simulink model "Aero_basic_tests"  (R2025a)
settings: Solver=ode1  StartTime=0.0  StopTime=240  FixedStep=0.002  RelTol=1e-3  EnableMultiTasking=on
undefined symbols (not defined in the file or in its folder): HIL, repelem
libraries: quarc_library x5, simulink x2
settings Model: SimulationMode=external  ExtModeTrigDuration=5000  Creator=MLevis  LastModifiedBy=e82540u
settings SolverCC: AlgebraicLoopSolver=TrustRegion  PositivePriorityOrder=on
settings DataIOCC: LimitDataPoints=on  SaveFormat=Array  ReturnWorkspaceOutputs=off
settings DebuggingCC: SolverPrmCheckMsg=warning  UnconnectedInputMsg=warning  UnconnectedOutputMsg=warning  UnconnectedLineMsg=warning  SFUnexpectedBacktrackingDiag=warning  SFNoUnconditionalDefaultTransitionDiag=warning  SFExecutionAtInitializationDiag=none  ArithmeticOperatorsInVariantConditions=warning
settings ModelReferenceCC: PropagateSignalLabelsOutOfModel=off
settings SFSimCC: SimUseLocalCustomCode=off  CustomCodeUndefinedFunction=UseInterfaceOnly
settings RTWCC: SystemTargetFile=quarc_win64.tlc  TemplateMakefile=quarc_default_tmf  RTWUseLocalCustomCode=off  Toolchain=QUARC win64 | nmake (64-bit Windows)  BuildConfiguration=Faster Runs  GPUComputeCapability=3.5  Description=QUARC Win64 Target Using Toolchain
settings CodeAppCC: StateflowObjectComments=on
settings STFCustomTargetCC: SystemTargetFile=quarc_win64.tlc  MultiwordLength=2048.0  DynamicStringBufferSize=256.0  ConcurrentExecutionCompliant=on  UseToolchainInfoCompliant=on
settings GRTTargetCC: ExtMode=on  ExtModeMexFile=quarc_comm  TargetLangStandard=C89/C90 (ANSI)  ParMdlRefBuildCompliant=off  CompOptLevelCompliant=off  CombineOutputUpdateFcns=off  MatFileLogging=off  CPPClassGenCompliant=off  GRTInterface=on
settings ConfigComp: CovMetricSettings=dw  CovSaveCumulativeToWorkspaceVar=on  CovSaveSingleToWorkspaceVar=on  CovExternalEMLEnable=off  CovSFcnEnable=off

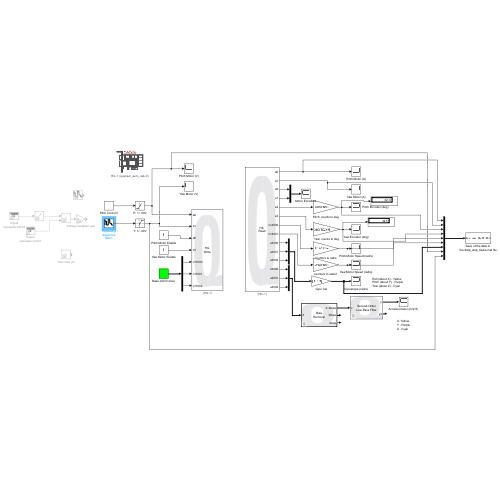
[thumbnail: Simulink's stored preview of the top-level diagram]
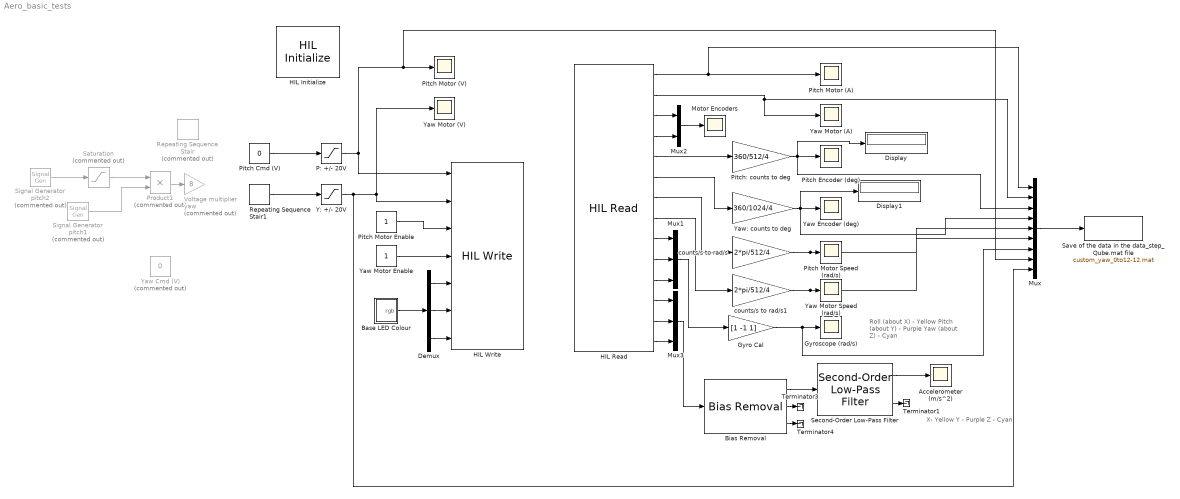
== system Aero_basic_tests ==
  note: Roll (about X) - Yellow
      | Pitch (about Y) - Purple
      | Yaw (about Z) - Cyan
  note: X- Yellow
      | Y - Purple
      | Z - Cyan
  Accelerometer (m/s^2) : Scope
      settings: DataLoggingVariableName=ScopeData10  DataLoggingSaveFormat=Array
  Base LED Colour : Subsystem  mask(Color Constant){color=[0 1 0]}
      mask help: Outputs a constant RGB color value.
      mask init:
      | rgb = get_param(gcbh, 'color');
      | if numel(color) ~= 3
      |     rgb = [0 0 0];
      | end
      | set_param(gcbh, 'MaskDisplay', ['patch([-0.02 -0.02 1.02 1.02], [-0.02 1.02 1.02 -0.02], ', rgb, ');']);
      settings: OpenFcn=color_constant_properties('CurrentBlock', gcbh);
      mask Help: web(qc_get_block_help_path(gcb), '-helpbrowser');
      mask Display: patch([-0.02 -0.02 1.02 1.02], [-0.02 1.02 1.02 -0.02], [0 1 0]);
  Bias Removal : quarc_library/Discrete/Bias Removal  start_time=0  end_time=0.1  switch_id=0  sample_time=qc_get_step_size
      settings: SourceProductName=QUARC Targets
  Demux : Demux  Outputs=3
  Display : Display
      settings: Decimation=20
  Display1 : Display
      settings: Decimation=20
  Gyro Cal : Gain  Gain=[1 -1 1]
  Gyroscope (rad/s) : Scope
      settings: TimeSpan=10  ActiveDisplayYMinimum=-2  ActiveDisplayYMaximum=2  DataLoggingVariableName=ScopeData9  DataLoggingSaveFormat=Array
  HIL Initialize : quarc_library/Data Acquisition/Generic/Configuration/HIL Initialize  Priority=-99  object_name=HIL-1  board_type=quanser_aero_usb  board_number=0  board_options=""  exclusive=off  active=off  hardware_clocks=[0]  clock_modes=[]  initial_clock_frequencies=[]  set_clock_params_at_start=off  set_clock_params_at_switch_in=off  set_clock_frequencies_at_start=off  set_clock_frequencies_at_switch_in=off  analog_input_channels=[0:1]  analog_input_configurations=[]  analog_input_maximums=3  analog_input_minimums=-3  set_analog_input_params_at_start=off  set_analog_input_params_at_switch_in=off  analog_output_channels=[0:1]  analog_output_maximums=24  analog_output_minimums=-24  initial_analog_outputs=[0]  final_analog_outputs=[0]  watchdog_analog_outputs=[0]  set_analog_output_params_at_start=off  set_analog_output_params_at_switch_in=off  set_analog_outputs_at_start=on  set_analog_outputs_at_switch_in=off  set_analog_outputs_at_terminate=on  set_analog_outputs_at_switch_out=off  set_analog_outputs_on_watchdog=on  digital_input_channels=[]  digital_output_channels=[0:1]  digital_output_configuration=[]  initial_digital_outputs=[1]  final_digital_outputs=[0]  watchdog_digital_outputs=[0]  set_digital_output_params_at_start=off  set_digital_output_params_at_switch_in=off  set_digital_outputs_at_start=on  set_digital_outputs_at_switch_in=off  set_digital_outputs_at_terminate=on  set_digital_outputs_at_switch_out=off  set_digital_outputs_on_watchdog=on  encoder_channels=[0:3]  quadrature=[4]  encoder_filter_frequency=[]  initial_encoder_counts=[0]  set_encoder_params_at_start=off  set_encoder_params_at_switch_in=off  set_encoder_counts_at_start=on  set_encoder_counts_at_switch_in=off  pwm_channels=[]  pwm_modes=[]  pwm_frequency=[]  pwm_configuration=[]  pwm_alignment=[]  pwm_polarity=[]  pwm_leading_deadband=[]  pwm_trailing_deadband=[]  initial_pwm_outputs=[]  final_pwm_outputs=[]  watchdog_pwm_outputs=[]  set_pwm_params_at_start=off  set_pwm_params_at_switch_in=off  set_pwm_outputs_at_start=off  set_pwm_outputs_at_switch_in=off  set_pwm_outputs_at_terminate=off  set_pwm_outputs_at_switch_out=off  set_pwm_outputs_on_watchdog=off  other_output_channels=[11000:11002]  initial_other_outputs=[0 1 0]  final_other_outputs=[1 0 0]  watchdog_other_outputs=[0 0 1]  set_other_outputs_at_start=on  set_other_outputs_at_switch_in=off  set_other_outputs_at_terminate=on  set_other_outputs_at_switch_out=off  set_other_outputs_on_watchdog=on
  HIL Read : quarc_library/Data Acquisition/Generic/Immediate I//O/HIL Read  object_name=HIL-1  analog_channels=[0:1]  encoder_channels=[0:3]  digital_channels=[]  other_channels=[14000:14001 3000:3002 4000:4002]  sample_time=qc_get_step_size  active=on  vector_output=off  data_type_mode=Inherit via back propagation  encoder_data_type=double  digital_data_type=boolean
  HIL Write : quarc_library/Data Acquisition/Generic/Immediate I//O/HIL Write  object_name=HIL-1  analog_channels=[0:1]  pwm_channels=[]  digital_channels=[0:1]  other_channels=[11000:11002]  sample_time=-1  active=off  vector_input=off
  Motor Encoders : Scope
      settings: ActiveDisplayYMinimum=-500000  ActiveDisplayYMaximum=0  DataLoggingVariableName=ScopeData2  DataLoggingSaveFormat=Array
  Mux : Mux  Inputs=9
  Mux1 : Mux  Inputs=3
  Mux2 : Mux  Inputs=2
  Mux3 : Mux  Inputs=3
  P: +/- 20V : Saturate  UpperLimit=20  LowerLimit=-20
  Pitch Cmd (V) : Constant  Value=0
  Pitch Encoder (deg) : Scope
      settings: ActiveDisplayYMinimum=-3.4716796874999991  ActiveDisplayYMaximum=31.2451171875  DataLoggingVariableName=ScopeData3  DataLoggingSaveFormat=Array
  Pitch Motor (A) : Scope
      settings: TimeSpan=10  ActiveDisplayYMinimum=-2.5  ActiveDisplayYMaximum=2.5  DataLoggingSaveFormat=Array
  Pitch Motor (V) : Scope
      settings: TimeSpan=10  ActiveDisplayYMinimum=-27.29039769480438  ActiveDisplayYMaximum=26.281397327441944  DataLoggingVariableName=ScopeData5  DataLoggingSaveFormat=Array
  Pitch Motor Enable : Constant
  Pitch Motor Speed (rad/s) : Scope
      settings: TimeSpan=10  ActiveDisplayYMinimum=-1000  ActiveDisplayYMaximum=1000  DataLoggingSaveFormat=Array
  Pitch: counts to deg : Gain  Gain=360/512/4
  Product1 : Product  Commented=on
  Repeating Sequence Stair : simulink/Sources/Repeating Sequence Stair  Commented=on  OutValues=repelem([0 1 2 3 4 5 6 7 8 9 10],5000)  tsamp=0.002  OutMin=[]  OutMax=[]  OutDataTypeStr=double  OutputDataTypeScalingMode=double  OutDataType=fixdt(0,8)  ConRadixGroup=Best Precision: Vector-wise  OutScaling=2^-12
  Repeating Sequence Stair1 : simulink/Sources/Repeating Sequence Stair  OutValues=repelem(reshape([zeros(1,12); 1:12; zeros(1,12); -(1:12)], 1, []), 5/0.002)  tsamp=0.002  OutMin=[]  OutMax=[]  OutDataTypeStr=double  OutputDataTypeScalingMode=double  OutDataType=fixdt(0,8)  ConRadixGroup=Best Precision: Vector-wise  OutScaling=2^-12
  Saturation : Saturate  Commented=on  UpperLimit=1  LowerLimit=0
  Save of the data in the data_step_Qube.mat file : ToFile  Filename=custom_yaw_0to12-12.mat  MatrixName=data0
  Second-Order Low-Pass Filter : quarc_library/Continuous/Second-Order Low-Pass Filter  params_source=Internal (dialog parameters)  input_width=2*pi*15  input_zeta=1  input_init=0
  Signal Generator pitch1 : SignalGenerator  Commented=on  WaveForm=square  Frequency=0.025
  Signal Generator pitch2 : SignalGenerator  Commented=on  WaveForm=square  Frequency=0.05
  Terminator1 : Terminator
  Terminator3 : Terminator
  Terminator4 : Terminator
  Voltage multiplier yaw : Gain  Commented=on  Gain=8
  Y: +/- 20V : Saturate  UpperLimit=20  LowerLimit=-20
  Yaw Cmd (V) : Constant  Commented=on  Value=0
  Yaw Encoder (deg) : Scope
      settings: TimeSpan=10  ActiveDisplayYMinimum=8641.614990234375  ActiveDisplayYMaximum=9752.222900390625  DataLoggingVariableName=ScopeData4  DataLoggingSaveFormat=Array
  Yaw Motor (A) : Scope
      settings: TimeSpan=10  ActiveDisplayYMinimum=0.20826514411333658  ActiveDisplayYMaximum=0.24554531021006348  DataLoggingVariableName=ScopeData7  DataLoggingSaveFormat=Array
  Yaw Motor (V) : Scope
      settings: TimeSpan=10  ActiveDisplayYMinimum=-25  ActiveDisplayYMaximum=25  DataLoggingVariableName=ScopeData6  DataLoggingSaveFormat=Array
  Yaw Motor Enable : Constant
  Yaw Motor Speed (rad/s) : Scope
      settings: TimeSpan=10  ActiveDisplayYMinimum=-100000  ActiveDisplayYMaximum=100000  DataLoggingVariableName=ScopeData8  DataLoggingSaveFormat=Array
  Yaw: counts to deg : Gain  Gain=360/1024/4
  counts/s to rad/s : Gain  Gain=2*pi/512/4
  counts/s to rad/s1 : Gain  Gain=2*pi/512/4
  wires:
  Base LED Colour/1(rgb) -> Demux/1
  Demux/1 -> HIL Write/5
  Demux/2 -> HIL Write/6
  Demux/3 -> HIL Write/7
  HIL Read/4 -> Mux2/2
  HIL Read/3 -> Mux2/1
  HIL Read/5 -> Pitch: counts to deg/1
  HIL Read/6 -> Yaw: counts to deg/1
  Mux2/1 -> Motor Encoders/1
  Pitch: counts to deg/1 -> Mux/3, Display/1, Pitch Encoder (deg)/1
  Y: +/- 20V/1 -> Mux/9, Yaw Motor (V)/1, HIL Write/2
  P: +/- 20V/1 -> HIL Write/1, Mux/8, Pitch Motor (V)/1
  HIL Read/1 -> Mux/1, Pitch Motor (A)/1
  HIL Read/2 -> Mux/2, Yaw Motor (A)/1
  Pitch Motor Enable/1 -> HIL Write/3
  Yaw Motor Enable/1 -> HIL Write/4
  HIL Read/11 -> Mux1/3
  HIL Read/9 -> Mux1/1
  HIL Read/10 -> Mux1/2
  Mux1/1 -> Gyro Cal/1
  HIL Read/13 -> Mux3/2
  HIL Read/12 -> Mux3/1
  HIL Read/14 -> Mux3/3
  Second-Order Low-Pass Filter/2 -> Terminator1/1
  Bias Removal/1 -> Second-Order Low-Pass Filter/1
  Mux3/1 -> Bias Removal/1
  Bias Removal/2 -> Terminator3/1
  Bias Removal/3 -> Terminator4/1
  Gyro Cal/1 -> Mux/7, Gyroscope (rad/s)/1
  Second-Order Low-Pass Filter/1 -> Accelerometer (m/s^2)/1
  HIL Read/7 -> counts/s to rad/s/1
  counts/s to rad/s/1 -> Mux/5, Pitch Motor Speed (rad/s)/1
  HIL Read/8 -> counts/s to rad/s1/1
  counts/s to rad/s1/1 -> Mux/6, Yaw Motor Speed (rad/s)/1
  Yaw: counts to deg/1 -> Mux/4, Display1/1, Yaw Encoder (deg)/1
  Mux/1 -> Save of the data in the data_step_Qube.mat file/1
  Signal Generator pitch2/1 -> Saturation/1
  Product1/1 -> Voltage multiplier yaw/1
  Signal Generator pitch1/1 -> Product1/2
  Saturation/1 -> Product1/1
  Pitch Cmd (V)/1 -> P: +/- 20V/1
  Repeating Sequence Stair1/1 -> Y: +/- 20V/1

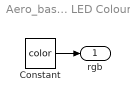
== system Aero_basic_tests/Base LED Colour ==
  Constant : Constant  Value=color
  rgb : Outport
  wires:
  Constant/1 -> rgb/1
